simulink model "SafeBeat_v1_step11_backup"  (R2019a)
settings: Solver=FixedStepDiscrete  StartTime=0.0  StopTime=10.0  FixedStep=0.027778  RelTol=1e-3
libraries: simulink x2, dsparch4 x1
settings Model: Creator=Admin  LastModifiedBy=Admin

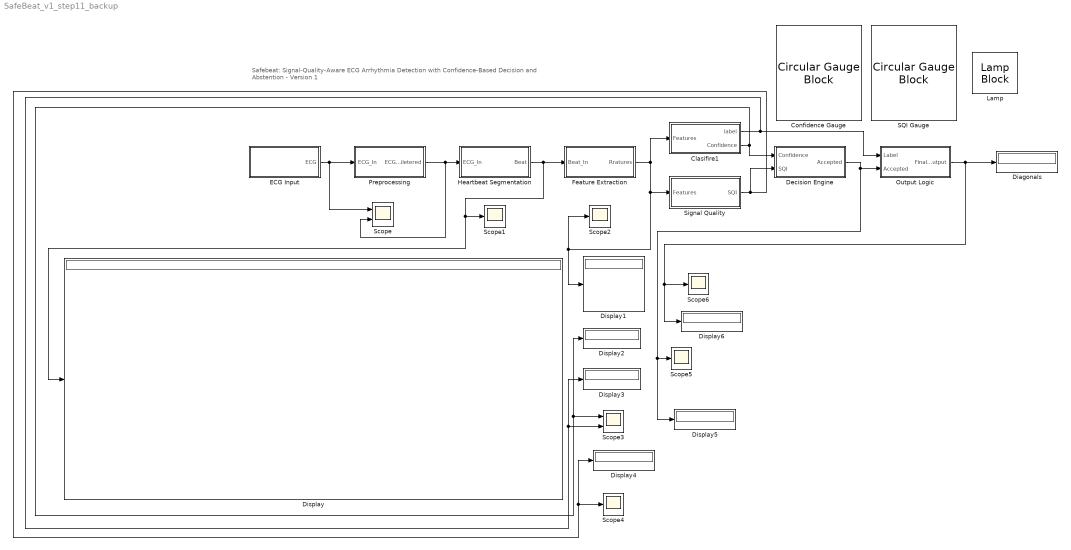
== system SafeBeat_v1_step11_backup ==
  note: Safebeat: Signal-Quality-Aware ECG Arrhythmia Detection with Confidence-Based Decision and Abstention - Version 1
  Clasifire1 : Subsystem
  Confidence Gauge : CircularGaugeBlock  ScaleMax=1
  Decision Engine : Subsystem
  "Diagonals " : Display
  Display{,1..6} (7 alike) : Display
  ECG Input : Subsystem
  Feature Extraction : Subsystem
  Heartbeat Segmentation : Subsystem
  Lamp : LampBlock
  Output Logic : Subsystem
  Preprocessing : Subsystem
  SQI Gauge : CircularGaugeBlock  ScaleMax=1
  Scope : Scope  NumInputPorts=2
  Scope{1..2,4..6} (5 alike) : Scope
  Scope3 : Scope  NumInputPorts=2
  Signal Quality : Subsystem
  wires:
  ECG Input/1(ECG) -> Preprocessing/1(ECG_In), Scope/1
  Preprocessing/1(ECG_Filetered) -> Heartbeat Segmentation/1(ECG_In), Scope/2
  Heartbeat Segmentation/1("Beat ") -> Feature Extraction/1(Beat_In), Display/1, Scope1/1
  Feature Extraction/1(Rratures) -> Clasifire1/1(Features), Signal Quality/1(Features), Display1/1, Scope2/1
  Clasifire1/2(Confidence) -> Scope3/1, Display2/1, Decision Engine/1(Confidence)
  Clasifire1/1(label) -> Scope3/2, Display3/1, Output Logic/1(Label)
  Signal Quality/1(SQI) -> Decision Engine/2(SQI), Scope4/1, Display4/1
  Decision Engine/1(Accepted) -> Output Logic/2(Accepted), Display5/1, Scope5/1
  Output Logic/1(FinalOutput) -> "Diagonals "/1, Scope6/1, Display6/1

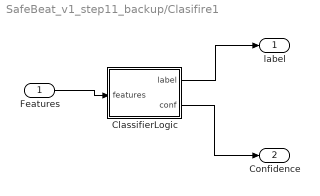
== system SafeBeat_v1_step11_backup/Clasifire1 ==
  Features : Inport
  ClassifierLogic : MATLAB Function  TreatAsAtomicUnit=on
  label : Outport
  Confidence : Outport  Port=2
  wires:
  ClassifierLogic/1(label) -> label/1
  Features/1 -> ClassifierLogic/1(features)
  ClassifierLogic/2(conf) -> Confidence/1

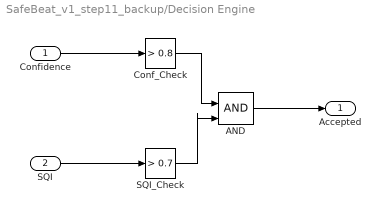
== system SafeBeat_v1_step11_backup/Decision Engine ==
  Confidence : Inport
  SQI : Inport  Port=2
  AND : Logic  IconShape=distinctive  AllPortsSameDT=off  OutDataTypeStr=boolean
  Conf_Check : simulink/Logic and Bit Operations/Compare To Constant  relop=>  const=0.8  OutDataTypeStr=boolean
  SQI_Check : simulink/Logic and Bit Operations/Compare To Constant  relop=>  const=0.7  OutDataTypeStr=boolean
  Accepted : Outport
  wires:
  Confidence/1 -> Conf_Check/1
  Conf_Check/1 -> AND/1
  SQI/1 -> SQI_Check/1
  SQI_Check/1 -> AND/2
  AND/1 -> Accepted/1

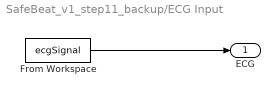
== system SafeBeat_v1_step11_backup/ECG Input ==
  "From Workspace " : FromWorkspace  VariableName=ecgSignal  SampleTime=0
  ECG : Outport
  wires:
  "From Workspace "/1 -> ECG/1

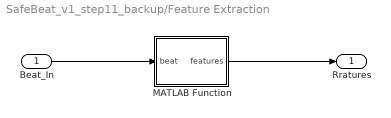
== system SafeBeat_v1_step11_backup/Feature Extraction ==
  Beat_In : Inport
  MATLAB Function : MATLAB Function  TreatAsAtomicUnit=on
  Rratures : Outport
  wires:
  MATLAB Function/1(features) -> Rratures/1
  Beat_In/1 -> MATLAB Function/1(beat)

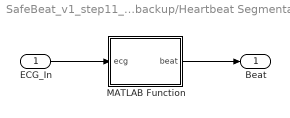
== system SafeBeat_v1_step11_backup/Heartbeat Segmentation ==
  ECG_In : Inport
  MATLAB Function : MATLAB Function  TreatAsAtomicUnit=on
  "Beat " : Outport
  wires:
  ECG_In/1 -> MATLAB Function/1(ecg)
  MATLAB Function/1(beat) -> "Beat "/1

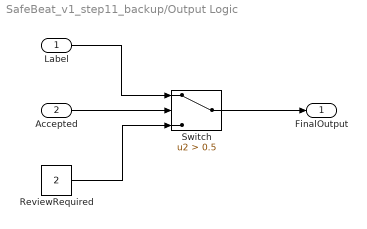
== system SafeBeat_v1_step11_backup/Output Logic ==
  Label : Inport
  Accepted : Inport  Port=2
  ReviewRequired : Constant  Value=2
  Switch : Switch  Criteria=u2 > Threshold  Threshold=0.5
  FinalOutput : Outport
  wires:
  Switch/1 -> FinalOutput/1
  Label/1 -> Switch/1
  Accepted/1 -> Switch/2
  ReviewRequired/1 -> Switch/3

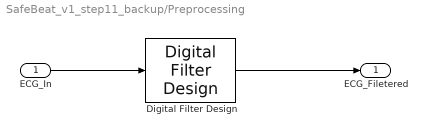
== system SafeBeat_v1_step11_backup/Preprocessing ==
  ECG_In : Inport
  Digital Filter Design : dsparch4/Digital Filter Design  mwdsp_browser_bugfix_var=off
  ECG_Filetered : Outport
  wires:
  ECG_In/1 -> Digital Filter Design/1
  Digital Filter Design/1 -> ECG_Filetered/1

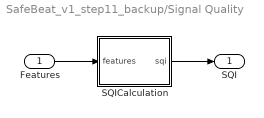
== system SafeBeat_v1_step11_backup/Signal Quality ==
  Features : Inport
  SQICalculation : MATLAB Function  TreatAsAtomicUnit=on
  SQI : Outport
  wires:
  Features/1 -> SQICalculation/1(features)
  SQICalculation/1(sqi) -> SQI/1

== matlab function SafeBeat_v1_step11_backup/Feature Extraction/MATLAB Function ==
  data: beat input; features output size=[4 1]
function features = fcn(beat)

meanVal = mean(beat);

stdVal = std(beat);

energyVal = sum(beat.^2);

peakVal = max(abs(beat));

features = [
    meanVal;
    stdVal;
    energyVal;
    peakVal
];

end

== matlab function SafeBeat_v1_step11_backup/Heartbeat Segmentation/MATLAB Function ==
  data: ecg input; beat output size=[250 1]
function beat = fcn(ecg)

persistent buffer

if isempty(buffer)
    buffer = zeros(250,1);
end

buffer = [buffer(2:end); ecg];

beat = buffer;

== matlab function SafeBeat_v1_step11_backup/Signal Quality/SQICalculation ==
  data: features input; sqi output double size=1
function sqi = calcSQI(features)

noiseMetric = features(2);

sqi = 1/(1 + noiseMetric);

end

== matlab function SafeBeat_v1_step11_backup/Clasifire1/ClassifierLogic ==
  data: features input; label output double size=1; conf output double size=1
function [label, conf] = classify(features)

energy = features(3);

if energy > 100

    label = 1;
    conf = 0.90;

else

    label = 0;
    conf = 0.85;

end

end
